simulink model "FOC"  (R2023a)
settings: Solver=ode3  StartTime=0.0  StopTime=20  FixedStep=1e-6  RelTol=1e-3
values from neighbouring files (symbols this model uses):
  inertialMoment = 0.0023    [Parameters.m]
  Ki_Id = Rs*omega_current    (= 5654.86677646)    [Parameters.m]
  Ki_Iq = Rs*omega_current    (= 5654.86677646)    [Parameters.m]
  Ki_T = inertialMoment*omega_speed^2    (= 90800.36049)    [Parameters.m]
  Kp_Id = Ld*omega_current    (= 4.71238898038)    [Parameters.m]
  Kp_Iq = Lq*omega_current    (= 4.71238898038)    [Parameters.m]
  Kp_T = 2*zeta*omega_speed*inertialMoment    (= 20.434175256)    [Parameters.m]
  magnetFlux = 0.02    [Parameters.m]
  polePairNumber = 2    [Parameters.m]
  Rs = 0.9    [Parameters.m]
  Udc = 70    [Parameters.m]
libraries: slpidlib x3, spsDCVoltageSourceLib x1, spsUniversalBridgeLib x1, mcbcontrolslib x1, spsPermanentMagnetSynchronousMachineLib x1, simulink x1, spsSVPWMGenerator2LevelLib x1, spsabctodq0Lib x1, sps_lib x1
settings Model: Creator=NGOC MAI  LastModifiedBy=NGOC MAI

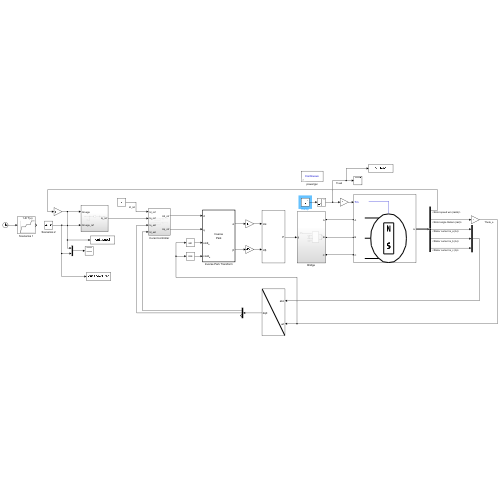
[thumbnail: Simulink's stored preview of the top-level diagram]
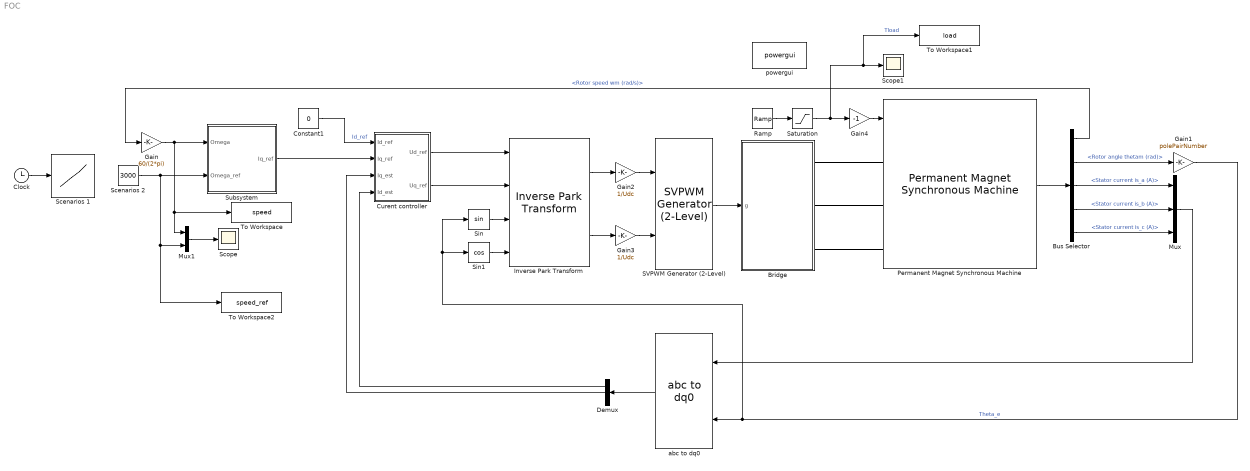
== system FOC ==
  Bridge : Subsystem
  Bus Selector : BusSelector  OutputSignals=Rotor speed wm (rad/s),Rotor angle thetam (rad),Stator current is_a (A),Stator current is_b (A),Stator current is_c (A)
  Clock : Clock
  Constant1 : Constant  Value=0
  Curent controller : Subsystem
  Demux : Demux  Outputs=3
  Gain : Gain  Gain=60/(2*pi)
  Gain1 : Gain  Gain=polePairNumber
  Gain2 : Gain  Gain=1/Udc
  Gain3 : Gain  Gain=1/Udc
  Gain4 : Gain  Gain=-1
  Inverse Park Transform : mcbcontrolslib/Inverse Park Transform  AxisAlignment=D-axis
      settings: LibrarySourceBlock=mcblib/Controls/Math Transforms/Inverse Park Transform
  Mux : Mux  Inputs=3
  Mux1 : Mux  Inputs=2
  Permanent Magnet Synchronous Machine : spsPermanentMagnetSynchronousMachineLib/Permanent Magnet Synchronous Machine  NbPhases=3  FluxDistribution=Sinusoidal  RotorType=Round  MechanicalLoad=Torque Tm  PresetModel=No  ShowDetailedParameters=on  MeasurementBus=off  Resistance=Rs  Inductance=8.5e-3  dqInductances=[8.5e-3,8.5e-3]  La=Ld  MachineConstant=Flux linkage established by magnets (V.s)  Flux=magnetFlux  VoltageCst=7.2552  TorqueCst=0.06  Flat=120  Mechanical=[inertialMoment 0.0004924 polePairNumber 0]  PolePairs=4  InitialConditions=[0,0, 0,0]  InitialConditions5ph=[0 0 0 0 0 0]  RefAngle=Aligned with phase A axis (original Park)  IterativeDiscreteModel=Trapezoidal non iterative  TsBlock=-1  TsPowergui=0
  Ramp : simulink/Sources/Ramp  slope=20  start=5  InitialOutput=0
  SVPWM Generator (2-Level) : spsSVPWMGenerator2LevelLib/SVPWM Generator (2-Level)  InputType=alpha-beta components  SwitchingPattern=Pattern #1  Fc=f  ParUref=[0.8 -30 50]  Ts=1e-5
  Saturation : Saturate  LowerLimit=-0.2
  Scenarios 1 : Lookup_n-D  NumberOfTableDimensions=1  BreakpointsForDimension1=[0, 2, 7, 9, 14, 16, 20]  Table=[0, 1500, 1500, 2000, 2000, 3000, 3000]  InternalRulePriority=Speed  RndMeth=Simplest
  Scenarios 2 : Constant  Value=3000
  Scope : Scope
  Scope1 : Scope
  Sin : Trigonometry
  Sin1 : Trigonometry  Operator=cos
  Subsystem : Subsystem
  To Workspace : ToWorkspace  VariableName=speed  SaveFormat=Timeseries  SampleTime=-1
  To Workspace1 : ToWorkspace  VariableName=load  SaveFormat=Timeseries  SampleTime=-1
  To Workspace2 : ToWorkspace  VariableName=speed_ref  SaveFormat=Timeseries  SampleTime=-1
  abc to dq0 : spsabctodq0Lib/abc to dq0  Alignment=Aligned with phase A axis
  powergui : sps_lib/powergui  Priority=1  SimulationMode=Continuous  SampleTime=50e-6  frequency=60  Iterations=50  frequencyindice=0  Pbase=100e6  ErrMax=1e-4  UnitsV=kV  UnitsW=MW  buscounter=0  FunctionMessages=off  echomessages=off  EnableUseOfTLC=off  CurrentSourceSwitches=off  DisableSnubberDevices=off  DisableRonSwitches=off  DisableVfSwitches=off  DisplayEquations=off  AutomaticDiscreteSolvers=off  SolverType=Tustin/Backward Euler (TBE)  Interpol=off  ExternalGateDelay=off  methode=off  Ts=100  x0status=blocks  SPID=on  SwTol=0  HookPort=off  NonlinearTolerance=1e-4  nMaxIteration=100  ContinueOnMaxIteration=off  RestoreLinks=warning  ResistiveCurrentMeasurement=off  Frange=[0:2:500]  Ylog=off  Xlog=on  ShowGrid=off  save=off  variable=ZData  structure=0  ZoomFFT=off  StartTime=0.0  cycles=1  DisplayStyle=1  fundamental=60  FreqAxis=off  MaxFrequency=1000  frequencyindicesteady=1  RmsSteady=1  display=off
  wires:
  Permanent Magnet Synchronous Machine/1 -> Bus Selector/1
  Bus Selector/2 -> Gain1/1  "<Rotor angle thetam (rad)>"
  Bus Selector/3 -> Mux/1  "<Stator current is_a (A)>"
  Bus Selector/4 -> Mux/2  "<Stator current is_b (A)>"
  Bus Selector/5 -> Mux/3  "<Stator current is_c (A)>"
  SVPWM Generator (2-Level)/1 -> Bridge/1(g)
  Mux/1 -> abc to dq0/1
  Gain1/1 -> Sin1/1, Sin/1, abc to dq0/2  "Theta_e"
  Constant1/1 -> Curent controller/1(Id_ref)  "Id_ref"
  Mux1/1 -> Scope/1
  Curent controller/1(Ud_ref) -> Inverse Park Transform/1
  Curent controller/2(Uq_ref) -> Inverse Park Transform/2
  Sin1/1 -> Inverse Park Transform/4
  Sin/1 -> Inverse Park Transform/3
  abc to dq0/1 -> Demux/1
  Demux/1 -> Curent controller/4(Id_est)
  Demux/2 -> Curent controller/3(Iq_est)
  Inverse Park Transform/1 -> Gain2/1
  Gain2/1 -> SVPWM Generator (2-Level)/1
  Inverse Park Transform/2 -> Gain3/1
  Gain3/1 -> SVPWM Generator (2-Level)/2
  Gain/1 -> Subsystem/1(Omega), To Workspace/1, Mux1/1
  Bus Selector/1 -> Gain/1  "<Rotor speed wm (rad/s)>"
  Subsystem/1(Iq_ref) -> Curent controller/2(Iq_ref)
  Saturation/1 -> Gain4/1, To Workspace1/1, Scope1/1  "Tload"
  Ramp/1 -> Saturation/1
  Clock/1 -> Scenarios 1/1
  Gain4/1 -> Permanent Magnet Synchronous Machine/1
  Scenarios 2/1 -> Mux1/2, To Workspace2/1, Subsystem/2(Omega_ref)
  connections:
  Bridge/RConn1 -- Permanent Magnet Synchronous Machine/LConn1
  Bridge/RConn2 -- Permanent Magnet Synchronous Machine/LConn2
  Bridge/RConn3 -- Permanent Magnet Synchronous Machine/LConn3

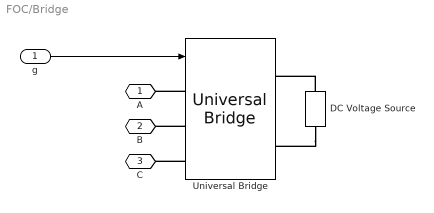
== system FOC/Bridge ==
  g : Inport
  DC Voltage Source : spsDCVoltageSourceLib/DC Voltage Source  Amplitude=Udc  Measurements=Voltage
  Universal Bridge : spsUniversalBridgeLib/Universal Bridge  Arms=3  SnubberResistance=1e5  SnubberCapacitance=inf  Device=IGBT / Diodes  Ron=1e-3  Lon=0  ForwardVoltages="[  0  0  ]"  ForwardVoltage=0  GTOparameters=[ 10e-6 , 20e-6 ]  IGBTparameters=[ 1e-6 , 2e-6 ]  Measurements=None  Measurements_2=None  converterType=Rectifier
  A : PMIOPort  Side=Right
  B : PMIOPort  Port=2  Side=Right
  C : PMIOPort  Port=3  Side=Right
  wires:
  g/1 -> Universal Bridge/1
  connections:
  Universal Bridge/LConn1 -- A/RConn1
  DC Voltage Source/LConn1 -- Universal Bridge/RConn2
  DC Voltage Source/RConn1 -- Universal Bridge/RConn1
  Universal Bridge/LConn2 -- B/RConn1
  Universal Bridge/LConn3 -- C/RConn1

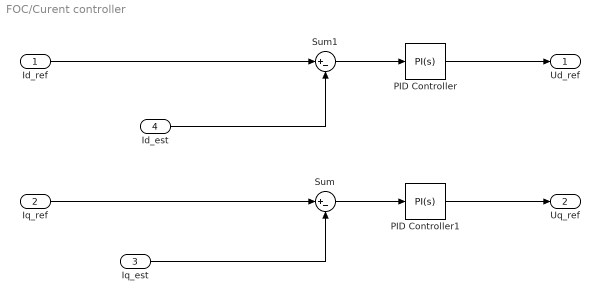
== system FOC/Curent controller ==
  Id_ref : Inport
  Iq_ref : Inport  Port=2
  Iq_est : Inport  Port=3
  Id_est : Inport  Port=4
  PID Controller : slpidlib/PID Controller  Controller=PI  Form=Parallel  TimeDomain=Continuous-time  UseExternalTs=off  SampleTime=-1  IntegratorMethod=Forward Euler  FilterMethod=Forward Euler  ControllerParametersSource=internal  P=Kp_Id  I=Ki_Id  UseKiTs=off  D=0  N=100  UseFilter=on  TunerSelectOption=Transfer Function Based (PID Tuner App)  InitialConditionSource=internal  InitialConditionForIntegrator=0  InitialConditionForFilter=0  DifferentiatorICPrevScaledInput=0  ExternalReset=none  TrackingMode=off  Kt=1  LimitOutput=off  SatLimitsSource=internal  UpperSaturationLimit=inf  LowerSaturationLimit=-inf  LinearizeAsGain=on  AntiWindupMode=none  Kb=1  LimitIntegrator=off  UpperIntegratorSaturationLimit=inf  LowerIntegratorSaturationLimit=-inf  POutMin=[]  POutMax=[]  IOutMin=[]  IOutMax=[]  DOutMin=[]  DOutMax=[]  NOutMin=[]  NOutMax=[]  SumOutMin=[]  SumOutMax=[]  SaturationOutMin=[]  SaturationOutMax=[]  PParamMin=[]  PParamMax=[]  IParamMin=[]  IParamMax=[]  DParamMin=[]  DParamMax=[]  NParamMin=[]  NParamMax=[]  KbParamMin=[]  KbParamMax=[]  KtParamMin=[]  KtParamMax=[]  KbOutMin=[]  KbOutMax=[]  KtOutMin=[]  KtOutMax=[]  IntegratorOutMin=[]  IntegratorOutMax=[]  FilterOutMin=[]  FilterOutMax=[]  SumI1OutMin=[]  SumI1OutMax=[]  SumI2OutMin=[]  SumI2OutMax=[]  SumI3OutMin=[]  SumI3OutMax=[]  SumI4OutMin=[]  SumI4OutMax=[]  SumDOutMin=[]  SumDOutMax=[]  DifferentiatorOutMin=[]  DifferentiatorOutMax=[]  FilterDiffOutCoefMin=[]  FilterDiffOutCoefMax=[]  ReciprocalOutMin=[]  ReciprocalOutMax=[]  SumDenOutMin=[]  SumDenOutMax=[]  SumNumOutMin=[]  SumNumOutMax=[]  DivideOutMin=[]  DivideOutMax=[]  UdiffTsProdOutMin=[]  UdiffTsProdOutMax=[]  NTsProdOutMin=[]  NTsProdOutMax=[]  UintegralTsProdOutMin=[]  UintegralTsProdOutMax=[]  UngainTsProdOutMin=[]  UngainTsProdOutMax=[]  ClampingZeroOutDataTypeStr=Inherit: Inherit via back propagation  ClampingZeroOutMin=[]  ClampingZeroOutMax=[]  FilterDenConstantOutDataTypeStr=Inherit: Inherit via back propagation  FilterDenConstantOutMin=[]  FilterDenConstantOutMax=[]  PCopyOutDataTypeStr=Inherit: Inherit via back propagation  PCopyOutMin=[]  PCopyOutMax=[]  NCopyOutDataTypeStr=Inherit: Inherit via back propagation  NCopyOutMin=[]  NCopyOutMax=[]  IntegratorContinuousStateAttributes=''  IntegratorStateMustResolveToSignalObject=off  IntegratorRTWStateStorageClass=Auto  FilterContinuousStateAttributes=''  FilterStateMustResolveToSignalObject=off  FilterRTWStateStorageClass=Auto  ParallelPVariant=InternalParameters  IdealPVariant=Disabled  IVariant=InternalParameters  DVariant=Disabled  IntegratorVariant=Continuous  SatVariant=Disabled  AWVariant=Passthrough  PCopyVariant=Disabled  TRVariant=Disabled  FdbkBlocksVariant=Forward  IdealPFdbkVariant=Disabled  SatFdbkVariant=Disabled  DerivativeFilterVariant=Disabled  NVariant=Disabled  NCopyVariant=Disabled_SignalSpec  FilterICVariant=Disabled  IntegratorICVariant=InternalICs  ExternalResetVariant=Disabled  TRSumVariant=Passthrough  SumFdbkVariant=Disabled  SumVariant=Sum_PI  TsampFilterVariant=InternalTs  TsampNgainVariant=Passthrough  TsampIntegralVariant=Disabled_SignalSpec  ExternalSaturationOutDataTypeStr=Inherit: Same as second input
  PID Controller1 : slpidlib/PID Controller  Controller=PI  Form=Parallel  TimeDomain=Continuous-time  UseExternalTs=off  SampleTime=-1  IntegratorMethod=Forward Euler  FilterMethod=Forward Euler  ControllerParametersSource=internal  P=Kp_Iq  I=Ki_Iq  UseKiTs=off  D=0  N=100  UseFilter=on  TunerSelectOption=Transfer Function Based (PID Tuner App)  InitialConditionSource=internal  InitialConditionForIntegrator=0  InitialConditionForFilter=0  DifferentiatorICPrevScaledInput=0  ExternalReset=none  TrackingMode=off  Kt=1  LimitOutput=off  SatLimitsSource=internal  UpperSaturationLimit=inf  LowerSaturationLimit=-inf  LinearizeAsGain=on  AntiWindupMode=none  Kb=1  LimitIntegrator=off  UpperIntegratorSaturationLimit=inf  LowerIntegratorSaturationLimit=-inf  POutMin=[]  POutMax=[]  IOutMin=[]  IOutMax=[]  DOutMin=[]  DOutMax=[]  NOutMin=[]  NOutMax=[]  SumOutMin=[]  SumOutMax=[]  SaturationOutMin=[]  SaturationOutMax=[]  PParamMin=[]  PParamMax=[]  IParamMin=[]  IParamMax=[]  DParamMin=[]  DParamMax=[]  NParamMin=[]  NParamMax=[]  KbParamMin=[]  KbParamMax=[]  KtParamMin=[]  KtParamMax=[]  KbOutMin=[]  KbOutMax=[]  KtOutMin=[]  KtOutMax=[]  IntegratorOutMin=[]  IntegratorOutMax=[]  FilterOutMin=[]  FilterOutMax=[]  SumI1OutMin=[]  SumI1OutMax=[]  SumI2OutMin=[]  SumI2OutMax=[]  SumI3OutMin=[]  SumI3OutMax=[]  SumI4OutMin=[]  SumI4OutMax=[]  SumDOutMin=[]  SumDOutMax=[]  DifferentiatorOutMin=[]  DifferentiatorOutMax=[]  FilterDiffOutCoefMin=[]  FilterDiffOutCoefMax=[]  ReciprocalOutMin=[]  ReciprocalOutMax=[]  SumDenOutMin=[]  SumDenOutMax=[]  SumNumOutMin=[]  SumNumOutMax=[]  DivideOutMin=[]  DivideOutMax=[]  UdiffTsProdOutMin=[]  UdiffTsProdOutMax=[]  NTsProdOutMin=[]  NTsProdOutMax=[]  UintegralTsProdOutMin=[]  UintegralTsProdOutMax=[]  UngainTsProdOutMin=[]  UngainTsProdOutMax=[]  ClampingZeroOutDataTypeStr=Inherit: Inherit via back propagation  ClampingZeroOutMin=[]  ClampingZeroOutMax=[]  FilterDenConstantOutDataTypeStr=Inherit: Inherit via back propagation  FilterDenConstantOutMin=[]  FilterDenConstantOutMax=[]  PCopyOutDataTypeStr=Inherit: Inherit via back propagation  PCopyOutMin=[]  PCopyOutMax=[]  NCopyOutDataTypeStr=Inherit: Inherit via back propagation  NCopyOutMin=[]  NCopyOutMax=[]  IntegratorContinuousStateAttributes=''  IntegratorStateMustResolveToSignalObject=off  IntegratorRTWStateStorageClass=Auto  FilterContinuousStateAttributes=''  FilterStateMustResolveToSignalObject=off  FilterRTWStateStorageClass=Auto  ParallelPVariant=InternalParameters  IdealPVariant=Disabled  IVariant=InternalParameters  DVariant=Disabled  IntegratorVariant=Continuous  SatVariant=Disabled  AWVariant=Passthrough  PCopyVariant=Disabled  TRVariant=Disabled  FdbkBlocksVariant=Forward  IdealPFdbkVariant=Disabled  SatFdbkVariant=Disabled  DerivativeFilterVariant=Disabled  NVariant=Disabled  NCopyVariant=Disabled_SignalSpec  FilterICVariant=Disabled  IntegratorICVariant=InternalICs  ExternalResetVariant=Disabled  TRSumVariant=Passthrough  SumFdbkVariant=Disabled  SumVariant=Sum_PI  TsampFilterVariant=InternalTs  TsampNgainVariant=Passthrough  TsampIntegralVariant=Disabled_SignalSpec  ExternalSaturationOutDataTypeStr=Inherit: Same as second input
  Sum : Sum  Inputs=|+-
  Sum1 : Sum  Inputs=|+-
  Ud_ref : Outport
  Uq_ref : Outport  Port=2
  wires:
  Iq_ref/1 -> Sum/1
  Sum/1 -> PID Controller1/1
  Id_ref/1 -> Sum1/1
  Sum1/1 -> PID Controller/1
  PID Controller/1 -> Ud_ref/1
  PID Controller1/1 -> Uq_ref/1
  Id_est/1 -> Sum1/2
  Iq_est/1 -> Sum/2

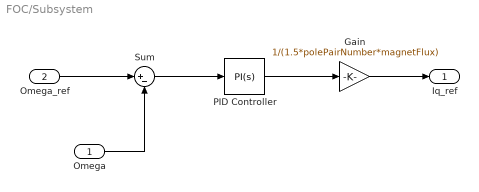
== system FOC/Subsystem ==
  Omega : Inport
  Omega_ref : Inport  Port=2
  Gain : Gain  Gain=1/(1.5*polePairNumber*magnetFlux)
  PID Controller : slpidlib/PID Controller  Controller=PI  Form=Parallel  TimeDomain=Continuous-time  UseExternalTs=off  SampleTime=-1  IntegratorMethod=Forward Euler  FilterMethod=Forward Euler  ControllerParametersSource=internal  P=Kp_T  I=Ki_T  UseKiTs=off  D=0  N=100  UseFilter=on  TunerSelectOption=Transfer Function Based (PID Tuner App)  InitialConditionSource=internal  InitialConditionForIntegrator=0  InitialConditionForFilter=0  DifferentiatorICPrevScaledInput=0  ExternalReset=none  TrackingMode=off  Kt=1  LimitOutput=on  SatLimitsSource=internal  UpperSaturationLimit=0.7  LowerSaturationLimit=-0.7  LinearizeAsGain=on  AntiWindupMode=clamping  Kb=1  LimitIntegrator=off  UpperIntegratorSaturationLimit=0.6  LowerIntegratorSaturationLimit=-0.6  POutMin=[]  POutMax=[]  IOutMin=[]  IOutMax=[]  DOutMin=[]  DOutMax=[]  NOutMin=[]  NOutMax=[]  SumOutMin=[]  SumOutMax=[]  SaturationOutMin=[]  SaturationOutMax=[]  PParamMin=[]  PParamMax=[]  IParamMin=[]  IParamMax=[]  DParamMin=[]  DParamMax=[]  NParamMin=[]  NParamMax=[]  KbParamMin=[]  KbParamMax=[]  KtParamMin=[]  KtParamMax=[]  KbOutMin=[]  KbOutMax=[]  KtOutMin=[]  KtOutMax=[]  IntegratorOutMin=[]  IntegratorOutMax=[]  FilterOutMin=[]  FilterOutMax=[]  SumI1OutMin=[]  SumI1OutMax=[]  SumI2OutMin=[]  SumI2OutMax=[]  SumI3OutMin=[]  SumI3OutMax=[]  SumI4OutMin=[]  SumI4OutMax=[]  SumDOutMin=[]  SumDOutMax=[]  DifferentiatorOutMin=[]  DifferentiatorOutMax=[]  FilterDiffOutCoefMin=[]  FilterDiffOutCoefMax=[]  ReciprocalOutMin=[]  ReciprocalOutMax=[]  SumDenOutMin=[]  SumDenOutMax=[]  SumNumOutMin=[]  SumNumOutMax=[]  DivideOutMin=[]  DivideOutMax=[]  UdiffTsProdOutMin=[]  UdiffTsProdOutMax=[]  NTsProdOutMin=[]  NTsProdOutMax=[]  UintegralTsProdOutMin=[]  UintegralTsProdOutMax=[]  UngainTsProdOutMin=[]  UngainTsProdOutMax=[]  ClampingZeroOutDataTypeStr=Inherit: Inherit via back propagation  ClampingZeroOutMin=[]  ClampingZeroOutMax=[]  FilterDenConstantOutDataTypeStr=Inherit: Inherit via back propagation  FilterDenConstantOutMin=[]  FilterDenConstantOutMax=[]  PCopyOutDataTypeStr=Inherit: Inherit via back propagation  PCopyOutMin=[]  PCopyOutMax=[]  NCopyOutDataTypeStr=Inherit: Inherit via back propagation  NCopyOutMin=[]  NCopyOutMax=[]  IntegratorContinuousStateAttributes=''  IntegratorStateMustResolveToSignalObject=off  IntegratorRTWStateStorageClass=Auto  FilterContinuousStateAttributes=''  FilterStateMustResolveToSignalObject=off  FilterRTWStateStorageClass=Auto  ParallelPVariant=InternalParameters  IdealPVariant=Disabled  IVariant=InternalParameters  DVariant=Disabled  IntegratorVariant=Continuous  SatVariant=Enabled  AWVariant=ContClampingParallel  PCopyVariant=Disabled  TRVariant=Disabled  FdbkBlocksVariant=Forward  IdealPFdbkVariant=Disabled  SatFdbkVariant=Disabled  DerivativeFilterVariant=Disabled  NVariant=Disabled  NCopyVariant=Disabled_SignalSpec  FilterICVariant=Disabled  IntegratorICVariant=InternalICs  ExternalResetVariant=Disabled  TRSumVariant=Passthrough  SumFdbkVariant=Disabled  SumVariant=Sum_PI  TsampFilterVariant=InternalTs  TsampNgainVariant=Passthrough  TsampIntegralVariant=Disabled_SignalSpec  ExternalSaturationOutDataTypeStr=Inherit: Same as second input
  Sum : Sum  Inputs=|+-
  Iq_ref : Outport
  wires:
  Omega/1 -> Sum/2
  Omega_ref/1 -> Sum/1
  Gain/1 -> Iq_ref/1
  Sum/1 -> PID Controller/1
  PID Controller/1 -> Gain/1
